simulink model "HybridPV"  (R2026b)
settings: Solver=VariableStepAuto
settings Model: Creator=Daksh  LastModifiedBy=Daksh

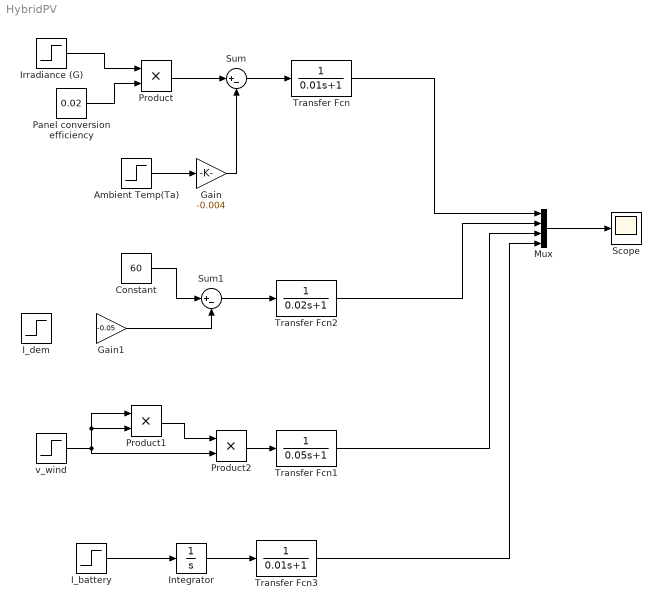
== system HybridPV ==
  Ambient Temp(Ta) : Step  Time=2  InitialValue=25  FinalValue=35  SampleTime=0
  Constant : Constant  Value=60
  Gain : Gain  Gain=-0.004
  Gain1 : Gain  Gain=-0.05
  I_battery : Step  Time=5  FinalValue=15  SampleTime=0
  I_dem : Step  Time=3  InitialValue=20  FinalValue=50  SampleTime=0
  Integrator : Integrator  InitialCondition=80
  Irradiance (G) : Step  Time=2  InitialValue=500  FinalValue=1000  SampleTime=0
  Mux : Mux
  Panel conversion efficiency : Constant  Value=0.02
  Product : Product
  Product1 : Product
  Product2 : Product
  Scope : Scope
      settings: ActiveDisplayYMinimum=-215.99999999999994  ActiveDisplayYMaximum=1944
  Sum : Sum  Inputs=|+-
  Sum1 : Sum  Inputs=|+-
  Transfer Fcn : TransferFcn  Denominator=[0.01 1]
  Transfer Fcn1 : TransferFcn  Denominator=[0.05 1]
  Transfer Fcn2 : TransferFcn  Denominator=[0.02 1]
  Transfer Fcn3 : TransferFcn  Denominator=[0.01 1]
  v_wind : Step  Time=4  InitialValue=8  FinalValue=12  SampleTime=0
  wires:
  Irradiance (G)/1 -> Product/1
  Panel conversion efficiency/1 -> Product/2
  Transfer Fcn/1 -> Mux/1
  Product/1 -> Sum/1
  Ambient Temp(Ta)/1 -> Gain/1
  Gain/1 -> Sum/2
  Sum/1 -> Transfer Fcn/1
  v_wind/1 -> Product2/2, Product1/2, Product1/1
  Product1/1 -> Product2/1
  Product2/1 -> Transfer Fcn1/1
  Transfer Fcn1/1 -> Mux/3
  Constant/1 -> Sum1/1
  Gain1/1 -> Sum1/2
  Sum1/1 -> Transfer Fcn2/1
  Transfer Fcn2/1 -> Mux/2
  I_battery/1 -> Integrator/1
  Integrator/1 -> Transfer Fcn3/1
  Transfer Fcn3/1 -> Mux/4
  Mux/1 -> Scope/1
